simulink model "StopTrigger_Bench_1b"  (R2025b)
settings: Solver=ode23t  StartTime=0.0  StopTime=10  MaxStep=0.01  RelTol=1e-3
model workspace (MAT data in the model file):
  Ald = 5743.49177499
  GLDR = 1.5
  GPT = 1
  Ipk = 4.37e-06
  R1 = 10000
  Rfix = 10000
  Rhyst = 47000
  Rin = 1000
  Tend = 0.1
  Tstart = 1
  Ttrip = 0.5
  Vcc = 5
  VrefL = 3.82978723404
  VrefP = 2.9375
  gam = 0.8
  seedN = 1
  sigN = 0.01
  t0 = 5
  tau = 0.25
  tauL = 0.05
libraries: fl_lib x38, nesl_utility x10, ee_lib x3, simulink x1
settings Model: Creator=davin  LastModifiedBy=davin
settings DataIOCC: SaveOutput=off  ReturnWorkspaceOutputs=off

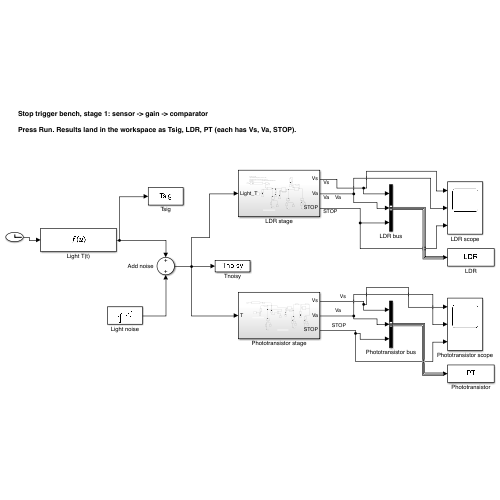
[thumbnail: Simulink's stored preview of the top-level diagram]
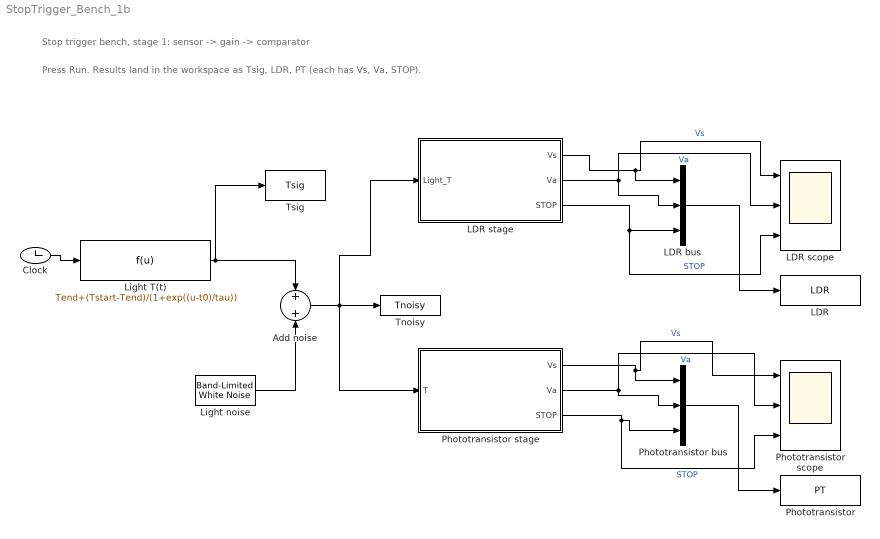
== system StopTrigger_Bench_1b ==
  note: Stop trigger bench, stage 1: sensor -> gain -> comparator
  note: Press Run. Results land in the workspace as Tsig, LDR, PT (each has Vs, Va, STOP).
  Add noise : Sum
  Clock : Clock
  LDR : ToWorkspace  VariableName=LDR  SaveFormat=Timeseries  SampleTime=-1
  LDR bus : BusCreator  Inputs=3
  LDR scope : Scope  NumInputPorts=3
      settings: Title=Sensor node Vs (falls when dark)  ActiveDisplayYMinimum=0  ActiveDisplayYMaximum=5  YLabel=Vs [V]
  LDR stage : Subsystem
  Light T(t) : Fcn  Expr=Tend+(Tstart-Tend)/(1+exp((u-t0)/tau))
  Light noise : simulink/Sources/Band-Limited White Noise  Cov=sigN^2*0.005  Ts=0.005  seed=[seedN]
  Phototransistor : ToWorkspace  VariableName=PT  SaveFormat=Timeseries  SampleTime=-1
  Phototransistor bus : BusCreator  Inputs=3
  Phototransistor scope : Scope  NumInputPorts=3
      settings: Title=Sensor node Vs (rises when dark)  ActiveDisplayYMinimum=0  ActiveDisplayYMaximum=5  YLabel=Vs [V]
  Phototransistor stage : Subsystem
  Tnoisy : ToWorkspace  VariableName=Tnoisy  SaveFormat=Timeseries  SampleTime=-1
  Tsig : ToWorkspace  VariableName=Tsig  SaveFormat=Timeseries  SampleTime=-1
  wires:
  Clock/1 -> Light T(t)/1
  LDR stage/1(Vs) -> LDR bus/1, LDR scope/1  "Vs"
  LDR stage/2(Va) -> LDR bus/2, LDR scope/2  "Va"
  LDR stage/3(STOP) -> LDR bus/3, LDR scope/3  "STOP"
  LDR bus/1 -> LDR/1
  Phototransistor stage/1(Vs) -> Phototransistor bus/1, Phototransistor scope/1  "Vs"
  Phototransistor stage/2(Va) -> Phototransistor bus/2, Phototransistor scope/2  "Va"
  Phototransistor stage/3(STOP) -> Phototransistor bus/3, Phototransistor scope/3  "STOP"
  Phototransistor bus/1 -> Phototransistor/1
  Light T(t)/1 -> Add noise/1, Tsig/1
  Light noise/1 -> Add noise/2
  Add noise/1 -> LDR stage/1(Light_T), Tnoisy/1, Phototransistor stage/1(T)

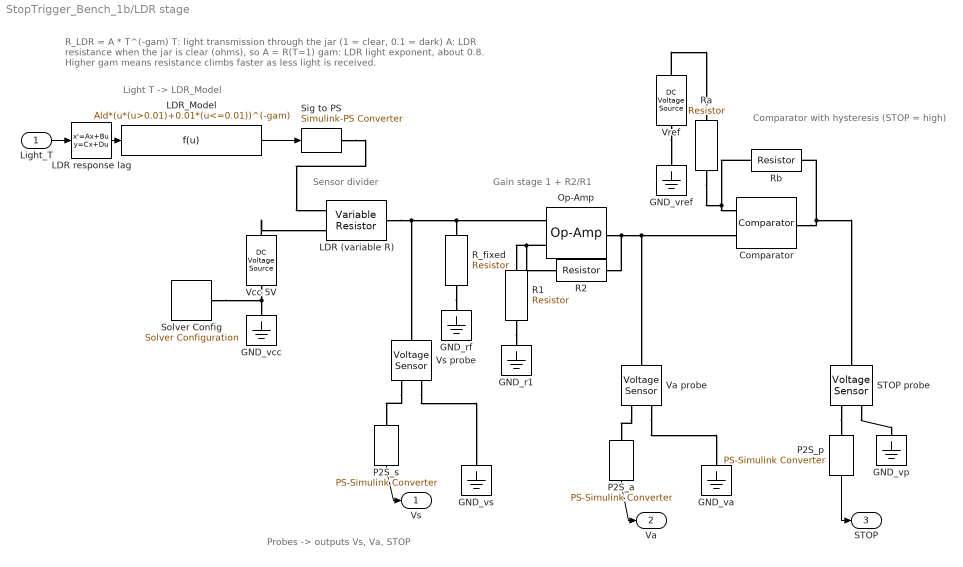
== system StopTrigger_Bench_1b/LDR stage ==
  note: R_LDR = A * T^(-gam)
      |
      | T: light transmission through the jar (1 = clear, 0.1 = dark)
      |
      | A: LDR resistance when the jar is clear (ohms), so A = R(T=1)
      |
      | gam: LDR light exponent, about 0.8. Higher gam means resistance climbs faster as less light is received.
  note: Light T -> LDR_Model
  note: Sensor divider
  note: Gain stage 1 + R2/R1
  note: Comparator with hysteresis (STOP = high)
  note: Probes -> outputs Vs, Va, STOP
  Light_T : Inport
  Comparator : ee_lib/Integrated Circuits/Comparator  V_OS=5 mV  C_IN=0 pF  V_OL=0 V  V_OH=5 V  R_OUT=50 Ohm  Delay=0 s
      settings: InternalSimscapePortConfiguration="{\"Bottom\":[],\"Left\":[{\"id\":\"p\",\"label\":\"+\",\"type\":\"foundation.electrical.electrical\"},{\"id\":\"n\",\"label\":\"-\",\"type\":\"foundation.electrical.electrical\"}],\"Right\":[{\"id\":\"J\",\"label\":\"\",\"type\":\"foundation.electrical.electrical\"}],\"Top\":[]}"
  GND_r1 : fl_lib/Electrical/Electrical Elements/Electrical Reference
  GND_rf : fl_lib/Electrical/Electrical Elements/Electrical Reference
  GND_va : fl_lib/Electrical/Electrical Elements/Electrical Reference
  GND_vcc : fl_lib/Electrical/Electrical Elements/Electrical Reference
  GND_vp : fl_lib/Electrical/Electrical Elements/Electrical Reference
  GND_vref : fl_lib/Electrical/Electrical Elements/Electrical Reference
  GND_vs : fl_lib/Electrical/Electrical Elements/Electrical Reference
  LDR (variable R) : fl_lib/Electrical/Electrical Elements/Variable Resistor  Rmin=0 Ohm  thermalEnable=false  thermal_mass=1 J/K  i_specify=off  i_priority=None  i=0 A  i_nominal_specify=off  i_nominal_value=1  i_nominal_unit=A  v_specify=off  v_priority=None  v=0 V  v_nominal_specify=off  v_nominal_value=1  v_nominal_unit=V  T_specify=off  T_priority=None  T=300 K  T_nominal_specify=off  T_nominal_value=1  T_nominal_unit=K
  LDR response lag : StateSpace  A=-1/tauL  B=1/tauL  D=0  InitialCondition=Tstart
  LDR_Model : Fcn  Expr=Ald*(u*(u>0.01)+0.01*(u<=0.01))^(-gam)
  Op-Amp : fl_lib/Electrical/Electrical Elements/Op-Amp  outI_specify=off  outI_priority=None  outI=0 A  outI_nominal_specify=off  outI_nominal_value=1  outI_nominal_unit=A
  P2S_a : nesl_utility/PS-Simulink Converter  PhysicalDomain=network_engine_domain  SubClassName=ps_output  LeftPortType=input  RightPortType=output  PseudoPeriodic=off  Frequencies=[]  VectorFormat=inherit  Unit=inherit  AffineConversion=off
  P2S_p : nesl_utility/PS-Simulink Converter  PhysicalDomain=network_engine_domain  SubClassName=ps_output  LeftPortType=input  RightPortType=output  PseudoPeriodic=off  Frequencies=[]  VectorFormat=inherit  Unit=inherit  AffineConversion=off
  P2S_s : nesl_utility/PS-Simulink Converter  PhysicalDomain=network_engine_domain  SubClassName=ps_output  LeftPortType=input  RightPortType=output  PseudoPeriodic=off  Frequencies=[]  VectorFormat=inherit  Unit=inherit  AffineConversion=off
  R1 : fl_lib/Electrical/Electrical Elements/Resistor  R=R1 Ohm  i_specify=off  i_priority=None  i=0 A  i_nominal_specify=off  i_nominal_value=1  i_nominal_unit=A  v_specify=off  v_priority=None  v=0 V  v_nominal_specify=off  v_nominal_value=1  v_nominal_unit=V
  R2 : fl_lib/Electrical/Electrical Elements/Resistor  R=max((GLDR-1)*R1,1) Ohm  i_specify=off  i_priority=None  i=0 A  i_nominal_specify=off  i_nominal_value=1  i_nominal_unit=A  v_specify=off  v_priority=None  v=0 V  v_nominal_specify=off  v_nominal_value=1  v_nominal_unit=V
  R_fixed : fl_lib/Electrical/Electrical Elements/Resistor  R=Rfix Ohm  i_specify=off  i_priority=None  i=0 A  i_nominal_specify=off  i_nominal_value=1  i_nominal_unit=A  v_specify=off  v_priority=None  v=0 V  v_nominal_specify=off  v_nominal_value=1  v_nominal_unit=V
  Ra : fl_lib/Electrical/Electrical Elements/Resistor  R=Rin Ohm  i_specify=off  i_priority=None  i=0 A  i_nominal_specify=off  i_nominal_value=1  i_nominal_unit=A  v_specify=off  v_priority=None  v=0 V  v_nominal_specify=off  v_nominal_value=1  v_nominal_unit=V
  Rb : fl_lib/Electrical/Electrical Elements/Resistor  R=Rhyst Ohm  i_specify=off  i_priority=None  i=0 A  i_nominal_specify=off  i_nominal_value=1  i_nominal_unit=A  v_specify=off  v_priority=None  v=0 V  v_nominal_specify=off  v_nominal_value=1  v_nominal_unit=V
  STOP probe : fl_lib/Electrical/Electrical Sensors/Voltage Sensor
  Sig to PS : nesl_utility/Simulink-PS Converter  PhysicalDomain=network_engine_domain  SubClassName=ps_input  LeftPortType=input  RightPortType=output  PseudoPeriodic=off  Frequencies=[]  NoiseDistribution=none  NoiseParameters=[]  Unit=1  AffineConversion=off  FilteringAndDerivatives=provide  SimscapeFilterOrder=1  InputFilterTimeConstant=0.001  UdotUserProvided=0
  Solver Config : nesl_utility/Solver Configuration  PhysicalDomain=network_engine_domain  SubClassName=solver  LeftPortType=input  RightPortType=generic  Tones=[]  Harmonics=[]  SimulateNoise=off  Profile=off  UseLocalSampling=off  EnableSwitchedLinearOptims=on  FrequencyDomain=off  UseCCode=off  RelTol=0.001  AbsTol=0.001  MinStep=1e-09  ToWorkspace=off  RevertToSquareIcSolve=off  NumHomotopyIterations=100  PhasorMode=off  PhasorModeNumHarmonics=1  ConsistencySolver=NEWTON_XTOL_AFTER_FTOL  IndexReductionMethod=DerivativeReplacement  DoDC=off  ResidualTolerance=1e-09  ConsistencyTolSource=GLOBAL  ConsistencyAbsTol=0.001  ConsistencyRelTol=0.001  ConsistencyTolFactor=0.001  UseLocalSolver=off  LocalSolverChoice=NE_BACKWARD_EULER_ADVANCER  ResolveIndetEquations=on  FunctionEvalNumThread=1  LocalSolverSampleTime=0.001  DoFixedCost=off  MaxNonlinIter=3  MaxModeIter=2  ComputeImpulses=off  ImpulseIterations=2  LinearAlgebra=auto  LinearAlgebraNumThread=0  EquationFormulation=NE_TIME_EF  DelaysMemoryBudget=1024  AutomaticFiltering=on  FilteringTimeConstant=0.001  PartitionStorageMethod=AS_NEEDED  PartitionMemoryBudget=1024  PartitionMethod=ROBUST  MultibodyUseLocalSolver=off  MultibodyLocalSolverChoice=ODE1  MultibodyLocalSolverSampleTime=0.001
  Va probe : fl_lib/Electrical/Electrical Sensors/Voltage Sensor
  Vcc 5V : fl_lib/Electrical/Electrical Sources/DC Voltage Source  v0=Vcc V
  Vref : fl_lib/Electrical/Electrical Sources/DC Voltage Source  v0=VrefL V
  Vs probe : fl_lib/Electrical/Electrical Sensors/Voltage Sensor
  Vs : Outport
  Va : Outport  Port=2
  STOP : Outport  Port=3
  wires:
  LDR_Model/1 -> Sig to PS/1
  P2S_s/1 -> Vs/1
  P2S_a/1 -> Va/1
  P2S_p/1 -> STOP/1
  Light_T/1 -> LDR response lag/1
  LDR response lag/1 -> LDR_Model/1
  connections:
  Sig to PS/RConn1 -- LDR (variable R)/LConn1
  Vcc 5V/LConn1 -- LDR (variable R)/LConn2
  GND_vcc/LConn1 -- Vcc 5V/RConn1 -- Solver Config/RConn1
  R_fixed/LConn1 -- LDR (variable R)/RConn1 -- Vs probe/LConn1 -- Op-Amp/LConn1
  R_fixed/RConn1 -- GND_rf/LConn1
  Op-Amp/LConn2 -- R1/LConn1 -- R2/LConn1
  R1/RConn1 -- GND_r1/LConn1
  Op-Amp/RConn1 -- R2/RConn1 -- Va probe/LConn1 -- Comparator/LConn2
  Vref/LConn1 -- Ra/LConn1
  Vref/RConn1 -- GND_vref/LConn1
  Ra/RConn1 -- Rb/RConn1 -- Comparator/LConn1
  Rb/LConn1 -- STOP probe/LConn1 -- Comparator/RConn1
  Vs probe/RConn2 -- GND_vs/LConn1
  Va probe/RConn2 -- GND_va/LConn1
  STOP probe/RConn2 -- GND_vp/LConn1
  Vs probe/RConn1 -- P2S_s/LConn1
  Va probe/RConn1 -- P2S_a/LConn1
  STOP probe/RConn1 -- P2S_p/LConn1

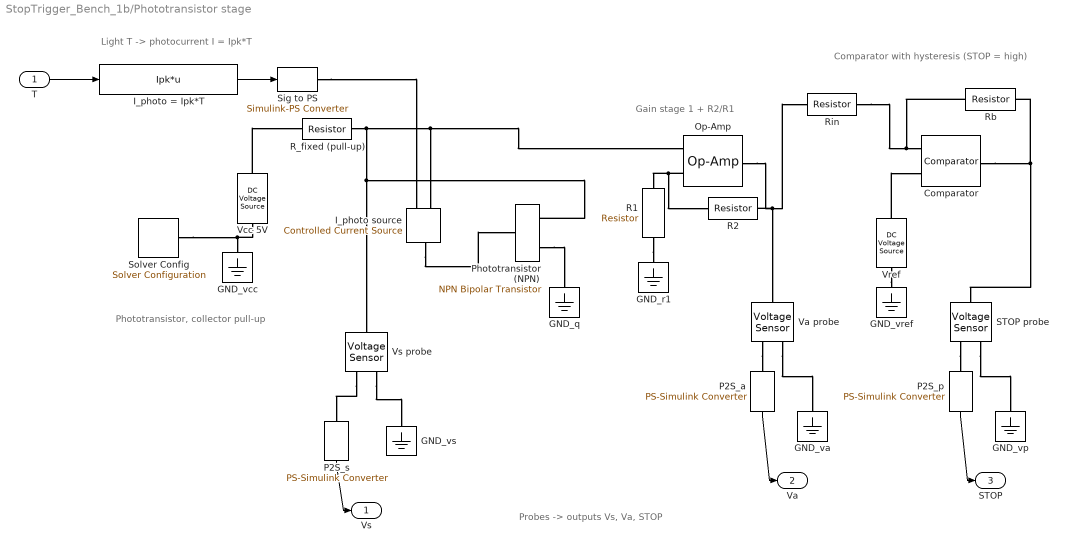
== system StopTrigger_Bench_1b/Phototransistor stage ==
  note: Light T -> photocurrent I = Ipk*T
  note: Phototransistor, collector pull-up
  note: Gain stage 1 + R2/R1
  note: Comparator with hysteresis (STOP = high)
  note: Probes -> outputs Vs, Va, STOP
  T : Inport
  Comparator : ee_lib/Integrated Circuits/Comparator  V_OS=5 mV  C_IN=0 pF  V_OL=0 V  V_OH=5 V  R_OUT=50 Ohm  Delay=0 s
      settings: InternalSimscapePortConfiguration="{\"Bottom\":[],\"Left\":[{\"id\":\"p\",\"label\":\"+\",\"type\":\"foundation.electrical.electrical\"},{\"id\":\"n\",\"label\":\"-\",\"type\":\"foundation.electrical.electrical\"}],\"Right\":[{\"id\":\"J\",\"label\":\"\",\"type\":\"foundation.electrical.electrical\"}],\"Top\":[]}"
  GND_q : fl_lib/Electrical/Electrical Elements/Electrical Reference
  GND_r1 : fl_lib/Electrical/Electrical Elements/Electrical Reference
  GND_va : fl_lib/Electrical/Electrical Elements/Electrical Reference
  GND_vcc : fl_lib/Electrical/Electrical Elements/Electrical Reference
  GND_vp : fl_lib/Electrical/Electrical Elements/Electrical Reference
  GND_vref : fl_lib/Electrical/Electrical Elements/Electrical Reference
  GND_vs : fl_lib/Electrical/Electrical Elements/Electrical Reference
  I_photo = Ipk*T : Fcn  Expr=Ipk*u
  I_photo source : fl_lib/Electrical/Electrical Sources/Controlled Current Source
  Op-Amp : fl_lib/Electrical/Electrical Elements/Op-Amp  outI_specify=off  outI_priority=None  outI=0 A  outI_nominal_specify=off  outI_nominal_value=1  outI_nominal_unit=A
  P2S_a : nesl_utility/PS-Simulink Converter  PhysicalDomain=network_engine_domain  SubClassName=ps_output  LeftPortType=input  RightPortType=output  PseudoPeriodic=off  Frequencies=[]  VectorFormat=inherit  Unit=inherit  AffineConversion=off
  P2S_p : nesl_utility/PS-Simulink Converter  PhysicalDomain=network_engine_domain  SubClassName=ps_output  LeftPortType=input  RightPortType=output  PseudoPeriodic=off  Frequencies=[]  VectorFormat=inherit  Unit=inherit  AffineConversion=off
  P2S_s : nesl_utility/PS-Simulink Converter  PhysicalDomain=network_engine_domain  SubClassName=ps_output  LeftPortType=input  RightPortType=output  PseudoPeriodic=off  Frequencies=[]  VectorFormat=inherit  Unit=inherit  AffineConversion=off
  Phototransistor (NPN) : ee_lib/Semiconductors & Converters/NPN Bipolar Transistor  parameterization=1  BF=100  IS=1e-14 A  VAF=200 V  hfe=100  hoe=50e-6 1/Ohm  Ic_h=1 mA  Vce_h=5 V  V1=0.55 V  I1=0.5 mA  BR=1  Tmeas=25 degC  RC=0.01 Ohm  RE=1e-4 Ohm  RB=1 Ohm  C_BC=5 pF  C_BE=5 pF  TF=0 us  TR=0 us  prmDatasheet=1  prmEquCoeff=1  hfe_T2=125  XTB=0  V1_T2=0.45 V  I1_T2=0.5 mA  Tmeas2=125 degC  EG=1.11 eV  XTI=3  TdeviceDatasheet=25 degC  TdeviceEquCoeff=25 degC  ec=1  ib_specify=off  ib_priority=None  ib=0 A  ib_nominal_specify=off  ib_nominal_value=1  ib_nominal_unit=A  ic_specify=off  ic_priority=None  ic=0 A  ic_nominal_specify=off  ic_nominal_value=1  ic_nominal_unit=A  vce_specify=off  vce_priority=None  vce=0 V  vce_nominal_specify=off  vce_nominal_value=1  vce_nominal_unit=V  vbe_specify=off  vbe_priority=None  vbe=0 V  vbe_nominal_specify=off  vbe_nominal_value=1  vbe_nominal_unit=V  Qbc_specify=off  Qbc_priority=High  Qbc=0 C  Qbc_nominal_specify=off  Qbc_nominal_value=1  Qbc_nominal_unit=uC  Qbe_specify=off  Qbe_priority=High  Qbe=0 C  Qbe_nominal_specify=off  Qbe_nominal_value=1  Qbe_nominal_unit=uC  thermal_network_parameterization=ee.enum.thermalNetworkTopology.junctionCase  Rth=[0, 10] K/W  Rth_Cauer=[1, 3, 10] K/W  Rth_Foster=[.08, .14, .22, .16] K/W  thermal_mass_parameterization=ee.enum.thermalNetwork.timeconstant  thermal_mass=[0, 1] J/K  thermal_mass_Cauer=[.1, .3, 1] J/K  thermal_mass_Foster=[.001, .005, .05, .5] J/K  thermal_time_constant=[0, 10] s  thermal_time_constant_Cauer=[1, 3, 10] s  thermal_time_constant_Foster=[7e-05, .0007, .01, .08] s  thermal_mass_initial_temperatures=[25, 25] degC  thermal_mass_initial_temperatures_Cauer=[25, 25, 25] degC  Tvec_initial_Foster=[25, 25, 25, 25] degC
      settings: InternalSimscapePortConfiguration="{\"Bottom\":[],\"Left\":[{\"id\":\"B\",\"label\":\"\",\"type\":\"foundation.electrical.electrical\"}],\"Right\":[{\"id\":\"C\",\"label\":\"\",\"type\":\"foundation.electrical.electrical\"},{\"id\":\"E\",\"label\":\"\",\"type\":\"foundation.electrical.electrical\"}],\"Top\":[]}"
  R1 : fl_lib/Electrical/Electrical Elements/Resistor  R=R1 Ohm  i_specify=off  i_priority=None  i=0 A  i_nominal_specify=off  i_nominal_value=1  i_nominal_unit=A  v_specify=off  v_priority=None  v=0 V  v_nominal_specify=off  v_nominal_value=1  v_nominal_unit=V
  R2 : fl_lib/Electrical/Electrical Elements/Resistor  R=max((GPT-1)*R1,1) Ohm  i_specify=off  i_priority=None  i=0 A  i_nominal_specify=off  i_nominal_value=1  i_nominal_unit=A  v_specify=off  v_priority=None  v=0 V  v_nominal_specify=off  v_nominal_value=1  v_nominal_unit=V
  R_fixed (pull-up) : fl_lib/Electrical/Electrical Elements/Resistor  R=Rfix Ohm  i_specify=off  i_priority=None  i=0 A  i_nominal_specify=off  i_nominal_value=1  i_nominal_unit=A  v_specify=off  v_priority=None  v=0 V  v_nominal_specify=off  v_nominal_value=1  v_nominal_unit=V
  Rb : fl_lib/Electrical/Electrical Elements/Resistor  R=Rhyst Ohm  i_specify=off  i_priority=None  i=0 A  i_nominal_specify=off  i_nominal_value=1  i_nominal_unit=A  v_specify=off  v_priority=None  v=0 V  v_nominal_specify=off  v_nominal_value=1  v_nominal_unit=V
  Rin : fl_lib/Electrical/Electrical Elements/Resistor  R=Rin Ohm  i_specify=off  i_priority=None  i=0 A  i_nominal_specify=off  i_nominal_value=1  i_nominal_unit=A  v_specify=off  v_priority=None  v=0 V  v_nominal_specify=off  v_nominal_value=1  v_nominal_unit=V
  STOP probe : fl_lib/Electrical/Electrical Sensors/Voltage Sensor
  Sig to PS : nesl_utility/Simulink-PS Converter  PhysicalDomain=network_engine_domain  SubClassName=ps_input  LeftPortType=input  RightPortType=output  PseudoPeriodic=off  Frequencies=[]  NoiseDistribution=none  NoiseParameters=[]  Unit=1  AffineConversion=off  FilteringAndDerivatives=provide  SimscapeFilterOrder=1  InputFilterTimeConstant=0.001  UdotUserProvided=0
  Solver Config : nesl_utility/Solver Configuration  PhysicalDomain=network_engine_domain  SubClassName=solver  LeftPortType=input  RightPortType=generic  Tones=[]  Harmonics=[]  SimulateNoise=off  Profile=off  UseLocalSampling=off  EnableSwitchedLinearOptims=on  FrequencyDomain=off  UseCCode=off  RelTol=0.001  AbsTol=0.001  MinStep=1e-09  ToWorkspace=off  RevertToSquareIcSolve=off  NumHomotopyIterations=100  PhasorMode=off  PhasorModeNumHarmonics=1  ConsistencySolver=NEWTON_XTOL_AFTER_FTOL  IndexReductionMethod=DerivativeReplacement  DoDC=off  ResidualTolerance=1e-09  ConsistencyTolSource=GLOBAL  ConsistencyAbsTol=0.001  ConsistencyRelTol=0.001  ConsistencyTolFactor=0.001  UseLocalSolver=off  LocalSolverChoice=NE_BACKWARD_EULER_ADVANCER  ResolveIndetEquations=on  FunctionEvalNumThread=1  LocalSolverSampleTime=0.001  DoFixedCost=off  MaxNonlinIter=3  MaxModeIter=2  ComputeImpulses=off  ImpulseIterations=2  LinearAlgebra=auto  LinearAlgebraNumThread=0  EquationFormulation=NE_TIME_EF  DelaysMemoryBudget=1024  AutomaticFiltering=on  FilteringTimeConstant=0.001  PartitionStorageMethod=AS_NEEDED  PartitionMemoryBudget=1024  PartitionMethod=ROBUST  MultibodyUseLocalSolver=off  MultibodyLocalSolverChoice=ODE1  MultibodyLocalSolverSampleTime=0.001
  Va probe : fl_lib/Electrical/Electrical Sensors/Voltage Sensor
  Vcc 5V : fl_lib/Electrical/Electrical Sources/DC Voltage Source  v0=Vcc V
  Vref : fl_lib/Electrical/Electrical Sources/DC Voltage Source  v0=VrefP V
  Vs probe : fl_lib/Electrical/Electrical Sensors/Voltage Sensor
  Vs : Outport
  Va : Outport  Port=2
  STOP : Outport  Port=3
  wires:
  T/1 -> I_photo = Ipk*T/1
  I_photo = Ipk*T/1 -> Sig to PS/1
  P2S_s/1 -> Vs/1
  P2S_a/1 -> Va/1
  P2S_p/1 -> STOP/1
  connections:
  Sig to PS/RConn1 -- I_photo source/RConn1
  Vcc 5V/LConn1 -- R_fixed (pull-up)/LConn1
  GND_vcc/LConn1 -- Vcc 5V/RConn1 -- Solver Config/RConn1
  Phototransistor (NPN)/RConn1 -- Op-Amp/LConn1 -- I_photo source/RConn2 -- R_fixed (pull-up)/RConn1 -- Vs probe/LConn1
  I_photo source/LConn1 -- Phototransistor (NPN)/LConn1
  Phototransistor (NPN)/RConn2 -- GND_q/LConn1
  R1/LConn1 -- Op-Amp/LConn2 -- R2/LConn1
  R1/RConn1 -- GND_r1/LConn1
  R2/RConn1 -- Op-Amp/RConn1 -- Rin/LConn1 -- Va probe/LConn1
  Comparator/LConn1 -- Rin/RConn1 -- Rb/RConn1
  Comparator/RConn1 -- Rb/LConn1 -- STOP probe/LConn1
  Vref/LConn1 -- Comparator/LConn2
  Vref/RConn1 -- GND_vref/LConn1
  Vs probe/RConn2 -- GND_vs/LConn1
  Va probe/RConn2 -- GND_va/LConn1
  STOP probe/RConn2 -- GND_vp/LConn1
  Vs probe/RConn1 -- P2S_s/LConn1
  Va probe/RConn1 -- P2S_a/LConn1
  STOP probe/RConn1 -- P2S_p/LConn1
